simulink model "boost_converter_PID"  (R2026a)
settings: Solver=ode15s  StopTime=0.5  RelTol=1e-6  AbsTol=1e-9
undefined symbols (not defined in the file): C, L, rL, Rload, Vin, Vref
libraries: slpidlib x1
settings Model: Creator=akash  LastModifiedBy=akash

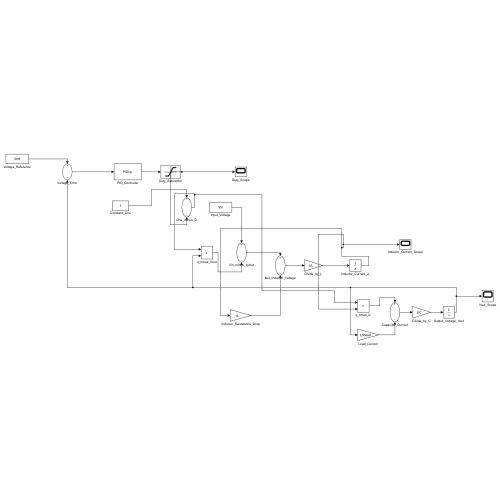
[thumbnail: Simulink's stored preview of the top-level diagram]
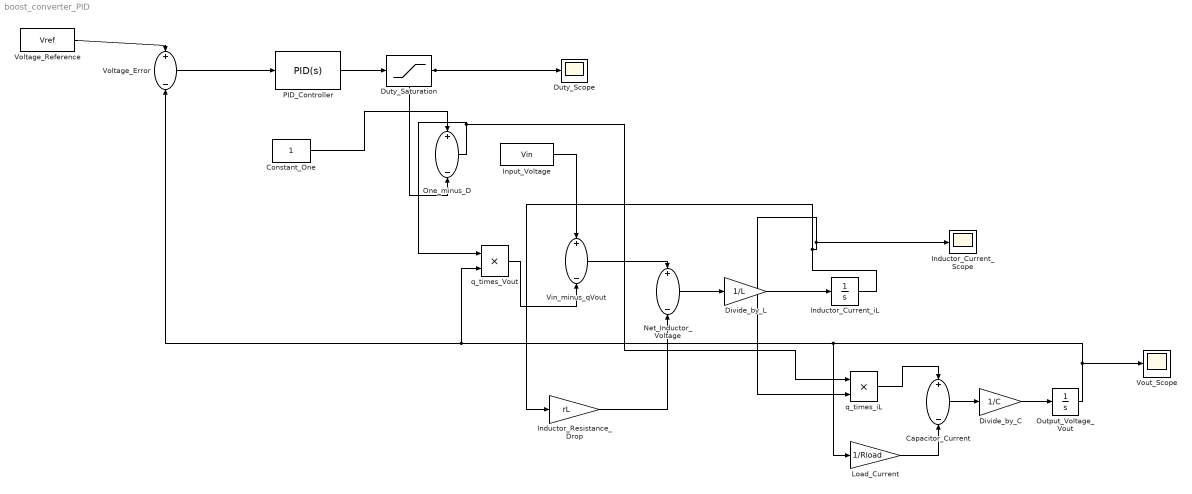
== system boost_converter_PID ==
  Capacitor_Current : Sum  Inputs=+-
  Constant_One : Constant
  Divide_by_C : Gain  Gain=1/C
  Divide_by_L : Gain  Gain=1/L
  Duty_Saturation : Saturate  UpperLimit=0.95  LowerLimit=0
  Duty_Scope : Scope
      settings: ActiveDisplayYMinimum=0.0502722540618149  ActiveDisplayYMaximum=0.55219596259392856
  Inductor_Current_Scope : Scope
      settings: ActiveDisplayYMinimum=-10.868178767595882  ActiveDisplayYMaximum=22.030482000766327
  Inductor_Current_iL : Integrator
  Inductor_Resistance_Drop : Gain  Gain=rL
  Input_Voltage : Constant  Value=Vin
  Load_Current : Gain  Gain=1/Rload
  Net_Inductor_Voltage : Sum  Inputs=+-
  One_minus_D : Sum  Inputs=+-
  Output_Voltage_Vout : Integrator
  PID_Controller : slpidlib/PID Controller  Controller=PID  Form=Parallel  TimeDomain=Continuous-time  UseExternalTs=off  SampleTime=-1  IntegratorMethod=Forward Euler  FilterMethod=Forward Euler  ControllerParametersSource=internal  P=0.01  I=0.5  UseKiTs=off  D=0  UseExternalDerivativeSource=off  N=100  UseFilter=on  TunerSelectOption=Transfer Function Based (PID Tuner App)  InitialConditionSource=internal  InitialConditionForIntegrator=0  InitialConditionForFilter=0  DifferentiatorICPrevScaledInput=0  ExternalReset=none  TrackingMode=off  Kt=1  LimitOutput=off  SatLimitsSource=internal  UpperSaturationLimit=inf  LowerSaturationLimit=-inf  LinearizeAsGain=on  AntiWindupMode=none  Kb=1  LimitIntegrator=off  UpperIntegratorSaturationLimit=inf  LowerIntegratorSaturationLimit=-inf  POutMin=[]  POutMax=[]  IOutMin=[]  IOutMax=[]  DOutMin=[]  DOutMax=[]  NOutMin=[]  NOutMax=[]  SumOutMin=[]  SumOutMax=[]  SaturationOutMin=[]  SaturationOutMax=[]  PParamMin=[]  PParamMax=[]  IParamMin=[]  IParamMax=[]  DParamMin=[]  DParamMax=[]  NParamMin=[]  NParamMax=[]  KbParamMin=[]  KbParamMax=[]  KtParamMin=[]  KtParamMax=[]  KbOutMin=[]  KbOutMax=[]  KtOutMin=[]  KtOutMax=[]  IntegratorOutMin=[]  IntegratorOutMax=[]  FilterOutMin=[]  FilterOutMax=[]  SumI1OutMin=[]  SumI1OutMax=[]  SumI2OutMin=[]  SumI2OutMax=[]  SumI3OutMin=[]  SumI3OutMax=[]  SumI4OutMin=[]  SumI4OutMax=[]  SumDOutMin=[]  SumDOutMax=[]  DifferentiatorOutMin=[]  DifferentiatorOutMax=[]  FilterDiffOutCoefMin=[]  FilterDiffOutCoefMax=[]  ReciprocalOutMin=[]  ReciprocalOutMax=[]  SumDenOutMin=[]  SumDenOutMax=[]  SumNumOutMin=[]  SumNumOutMax=[]  DivideOutMin=[]  DivideOutMax=[]  UdiffTsProdOutMin=[]  UdiffTsProdOutMax=[]  NTsProdOutMin=[]  NTsProdOutMax=[]  UintegralTsProdOutMin=[]  UintegralTsProdOutMax=[]  UngainTsProdOutMin=[]  UngainTsProdOutMax=[]  ClampingZeroOutDataTypeStr=Inherit: Inherit via back propagation  ClampingZeroOutMin=[]  ClampingZeroOutMax=[]  FilterDenConstantOutDataTypeStr=Inherit: Inherit via back propagation  FilterDenConstantOutMin=[]  FilterDenConstantOutMax=[]  PCopyOutDataTypeStr=Inherit: Inherit via back propagation  PCopyOutMin=[]  PCopyOutMax=[]  NCopyOutDataTypeStr=Inherit: Inherit via back propagation  NCopyOutMin=[]  NCopyOutMax=[]  IntegratorContinuousStateAttributes=''  IntegratorStateMustResolveToSignalObject=off  IntegratorRTWStateStorageClass=Auto  FilterContinuousStateAttributes=''  FilterStateMustResolveToSignalObject=off  FilterRTWStateStorageClass=Auto  ParallelPVariant=InternalParameters  IdealPVariant=Disabled  IVariant=InternalParameters  DVariant=InternalParameters  IntegratorVariant=Continuous  SatVariant=Disabled  AWVariant=Passthrough  PCopyVariant=Disabled  TRVariant=Disabled  FdbkBlocksVariant=Forward  IdealPFdbkVariant=Disabled  SatFdbkVariant=Disabled  DerivativeFilterVariant=ContFilter  NVariant=InternalParameters  NCopyVariant=Disabled  FilterICVariant=InternalICsFilter  IntegratorICVariant=InternalICs  ExternalResetVariant=Disabled  TRSumVariant=Passthrough  SumFdbkVariant=Disabled  SumVariant=Sum_PID  TsampFilterVariant=InternalTs  TsampNgainVariant=Passthrough  TsampIntegralVariant=Disabled_SignalSpec  ExternalSaturationOutDataTypeStr=Inherit: Same as second input  DerivativeSourceVariant=ErrorSignal  PreIntVariant=InternalPreInt
  Vin_minus_qVout : Sum  Inputs=+-
  Voltage_Error : Sum  Inputs=+-
  Voltage_Reference : Constant  Value=Vref
  Vout_Scope : Scope
      settings: ActiveDisplayYMinimum=-4.9999534901090481  ActiveDisplayYMaximum=44.999581410981442
  q_times_Vout : Product  Inputs=**
  q_times_iL : Product  Inputs=**
  wires:
  Voltage_Reference/1 -> Voltage_Error/1
  Output_Voltage_Vout/1 -> Voltage_Error/2, q_times_Vout/2, Load_Current/1, Vout_Scope/1
  Voltage_Error/1 -> PID_Controller/1
  PID_Controller/1 -> Duty_Saturation/1
  Duty_Saturation/1 -> One_minus_D/2, Duty_Scope/1
  Constant_One/1 -> One_minus_D/1
  One_minus_D/1 -> q_times_Vout/1, q_times_iL/1
  Input_Voltage/1 -> Vin_minus_qVout/1
  q_times_Vout/1 -> Vin_minus_qVout/2
  Inductor_Current_iL/1 -> q_times_iL/2, Inductor_Current_Scope/1, Inductor_Resistance_Drop/1
  Vin_minus_qVout/1 -> Net_Inductor_Voltage/1
  Inductor_Resistance_Drop/1 -> Net_Inductor_Voltage/2
  Net_Inductor_Voltage/1 -> Divide_by_L/1
  Divide_by_L/1 -> Inductor_Current_iL/1
  q_times_iL/1 -> Capacitor_Current/1
  Load_Current/1 -> Capacitor_Current/2
  Capacitor_Current/1 -> Divide_by_C/1
  Divide_by_C/1 -> Output_Voltage_Vout/1
